simulink model "DAB1_1_2024b"  (R2024b)
settings: Solver=VariableStepAuto  StartTime=0.0  StopTime=10.0  RelTol=1e-3
libraries: spsVoltageMeasurementLib x12, spsMosfetLib x8, spsSeriesRLCBranchLib x3, spsCurrentMeasurementLib x3, spsLinearTransformerLib x1, spsDCVoltageSourceLib x1, spspowerguiLib x1
settings Model: Creator=Ashutosh  LastModifiedBy=Ashutosh

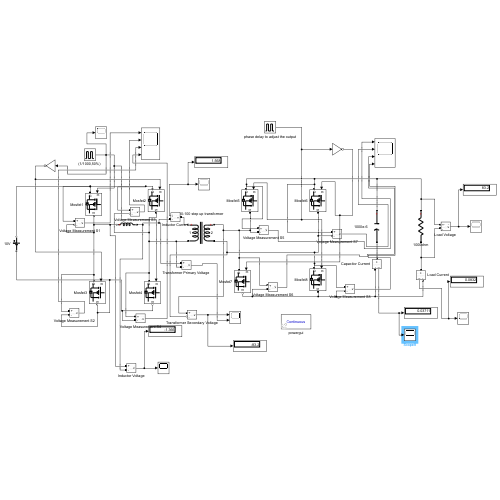
[thumbnail: Simulink's stored preview of the top-level diagram]
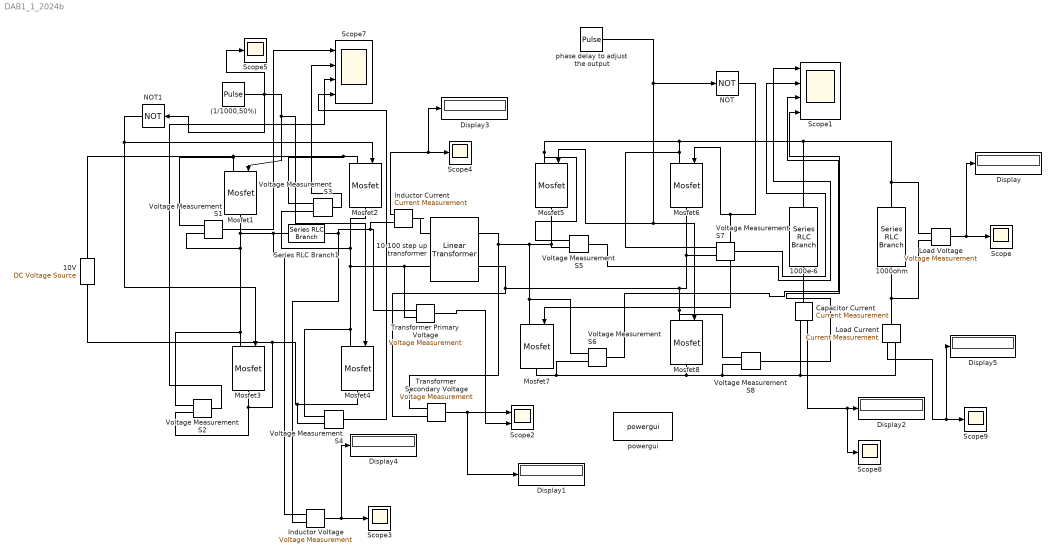
== system DAB1_1_2024b ==
  "(1/1000,50%) " : DiscretePulseGenerator  PulseType=Time based  Period=1/1000  PulseWidth=50
  10-100 step up transformer : spsLinearTransformerLib/Linear Transformer  UNITS=pu  NominalPower=[ 1000 1000 ]  winding1="[ 10  0  0 ]"  winding2="[ 100  0  0 ]"  ThreeWindings=off  winding3=[ 315e3 0.002 0.08 ]  RmLm=[ 500 500 ]  Measurements=None  DataType=off
  1000e-6 : spsSeriesRLCBranchLib/Series RLC Branch  LConnTagsString=__new0  RConnTagsString=__new0  BranchType=C  Resistance=1000  Inductance=1e-3  SetiL0=off  InitialCurrent=0  Capacitance=1000e-6  Setx0=off  InitialVoltage=0  Measurements=None
  1000ohm : spsSeriesRLCBranchLib/Series RLC Branch  LConnTagsString=__new0  RConnTagsString=__new0  BranchType=R  Resistance=1000  Inductance=1e-3  SetiL0=off  InitialCurrent=0  Capacitance=1e-6  Setx0=off  InitialVoltage=0  Measurements=None
  10V : spsDCVoltageSourceLib/DC Voltage Source  Amplitude=10  Measurements=None
  Capacitor Current : spsCurrentMeasurementLib/Current Measurement  PhasorSimulation=off  OutputType=Complex  PSBequivalent=0
  Display{,1..5} (6 alike) : Display
  Inductor Current : spsCurrentMeasurementLib/Current Measurement  PhasorSimulation=off  OutputType=Complex  PSBequivalent=0
  Inductor Voltage : spsVoltageMeasurementLib/Voltage Measurement  PhasorSimulation=off  OutputType=Complex  PSBequivalent=0
  "Load Current " : spsCurrentMeasurementLib/Current Measurement  PhasorSimulation=off  OutputType=Complex  PSBequivalent=0
  "Load Voltage " : spsVoltageMeasurementLib/Voltage Measurement  PhasorSimulation=off  OutputType=Complex  PSBequivalent=0
  Mosfet{1..8} (8 alike) : spsMosfetLib/Mosfet  Ron=0.1  Lon=0  Rd=0.01  Vfd=0  IC=0  Rs=1e5  Cs=inf  Measurements=off
  NOT : Logic  Operator=NOT  IconShape=distinctive  AllPortsSameDT=off  OutDataTypeStr=boolean
  NOT1 : Logic  Operator=NOT  IconShape=distinctive  AllPortsSameDT=off  OutDataTypeStr=boolean
  Scope{,3..5,8..9} (6 alike) : Scope
  Scope1 : Scope  NumInputPorts=4
  Scope2 : Scope  NumInputPorts=2
  Scope7 : Scope  NumInputPorts=4
  Series RLC Branch1 : spsSeriesRLCBranchLib/Series RLC Branch  LConnTagsString=__new0  RConnTagsString=__new0  BranchType=L  Resistance=1  Inductance=680e-6  SetiL0=off  InitialCurrent=0  Capacitance=1e-6  Setx0=off  InitialVoltage=0  Measurements=None
  "Transformer Primary Voltage " : spsVoltageMeasurementLib/Voltage Measurement  PhasorSimulation=off  OutputType=Complex  PSBequivalent=0
  Transformer Secondary Voltage : spsVoltageMeasurementLib/Voltage Measurement  PhasorSimulation=off  OutputType=Complex  PSBequivalent=0
  Voltage Measurement S{1..8} (8 alike) : spsVoltageMeasurementLib/Voltage Measurement  PhasorSimulation=off  OutputType=Complex  PSBequivalent=0
  phase delay to adjust the output : DiscretePulseGenerator  PulseType=Time based  Period=1/1000  PulseWidth=50  PhaseDelay=0.0834*(1/1000)
  powergui : spspowerguiLib/powergui  Priority=1  SimulationMode=Continuous  SampleTime=50e-6  frequency=60  Iterations=50  frequencyindice=0  Pbase=100e6  ErrMax=1e-4  UnitsV=kV  UnitsW=MW  buscounter=0  FunctionMessages=off  echomessages=off  EnableUseOfTLC=off  CurrentSourceSwitches=off  DisableSnubberDevices=off  DisableRonSwitches=off  DisableVfSwitches=off  DisplayEquations=off  AutomaticDiscreteSolvers=off  SolverType=Tustin/Backward Euler (TBE)  Interpol=off  ExternalGateDelay=off  methode=off  Ts=100  x0status=zero  SPID=on  SwTol=0  HookPort=off  NonlinearTolerance=1e-4  nMaxIteration=100  ContinueOnMaxIteration=off  RestoreLinks=warning  ResistiveCurrentMeasurement=off  Frange=[0:2:500]  Ylog=off  Xlog=on  ShowGrid=off  save=off  variable=ZData  structure=0  ZoomFFT=off  StartTime=0.0  cycles=1  DisplayStyle=1  fundamental=60  FreqAxis=off  MaxFrequency=1000  frequencyindicesteady=1  RmsSteady=1  display=off
  wires:
  Transformer Secondary Voltage/1 -> Scope2/1, Display1/1
  NOT/1 -> Mosfet7/1, Mosfet6/1
  NOT1/1 -> Mosfet2/1, Mosfet3/1
  "(1/1000,50%) "/1 -> Scope5/1, NOT1/1, Mosfet4/1, Mosfet1/1
  "Load Voltage "/1 -> Display/1, Scope/1
  phase delay to adjust the output/1 -> Mosfet8/1, Mosfet5/1, NOT/1
  Capacitor Current/1 -> Scope8/1, Display2/1
  Inductor Voltage/1 -> Scope3/1, Display4/1
  "Transformer Primary Voltage "/1 -> Scope2/2
  Voltage Measurement S5/1 -> Scope1/1
  Voltage Measurement S7/1 -> Scope1/2
  Voltage Measurement S6/1 -> Scope1/3
  Voltage Measurement S8/1 -> Scope1/4
  Voltage Measurement S1/1 -> Scope7/1
  Voltage Measurement S3/1 -> Scope7/2
  Voltage Measurement S2/1 -> Scope7/3
  Voltage Measurement S4/1 -> Scope7/4
  Inductor Current/1 -> Scope4/1, Display3/1
  "Load Current "/1 -> Scope9/1, Display5/1
  connections:
  10-100 step up transformer/RConn1 -- Transformer Secondary Voltage/LConn1 -- Voltage Measurement S6/LConn1 -- Mosfet7/LConn1 -- Voltage Measurement S5/LConn2 -- Mosfet5/RConn1
  Capacitor Current/RConn1 -- "Load Current "/RConn1 -- Voltage Measurement S8/LConn2 -- Mosfet8/RConn1 -- Voltage Measurement S6/LConn2 -- Mosfet7/RConn1
  10-100 step up transformer/RConn2 -- Transformer Secondary Voltage/LConn2 -- Voltage Measurement S8/LConn1 -- Mosfet8/LConn1 -- Mosfet6/RConn1 -- Voltage Measurement S7/LConn2
  Voltage Measurement S4/LConn1 -- Mosfet4/LConn1 -- "Transformer Primary Voltage "/LConn2 -- 10-100 step up transformer/LConn2 -- Voltage Measurement S3/LConn2 -- Mosfet2/RConn1
  Voltage Measurement S1/LConn1 -- Mosfet1/LConn1 -- 10V/RConn1 -- Voltage Measurement S3/LConn1 -- Mosfet2/LConn1
  Mosfet3/LConn1 -- Voltage Measurement S2/LConn1 -- Voltage Measurement S1/LConn2 -- Inductor Voltage/LConn1 -- Series RLC Branch1/LConn1 -- Mosfet1/RConn1
  1000ohm/LConn1 -- "Load Voltage "/LConn1 -- 1000e-6/LConn1 -- Voltage Measurement S5/LConn1 -- Mosfet5/LConn1 -- Voltage Measurement S7/LConn1 -- Mosfet6/LConn1
  Voltage Measurement S2/LConn2 -- Mosfet3/RConn1 -- 10V/LConn1 -- Mosfet4/RConn1 -- Voltage Measurement S4/LConn2
  Capacitor Current/LConn1 -- 1000e-6/RConn1
  Series RLC Branch1/RConn1 -- Inductor Voltage/LConn2 -- Inductor Current/RConn1 -- "Transformer Primary Voltage "/LConn1
  Inductor Current/LConn1 -- 10-100 step up transformer/LConn1
  1000ohm/RConn1 -- "Load Current "/LConn1 -- "Load Voltage "/LConn2
